simulink model "BESS_asset"  (R2026a)
settings: Solver=ode4  StopTime=inf  FixedStep=Tsim
model workspace (MATLAB code in the model file):
  | % Defaults for standalone use. In HPP.slx each instance k gets p.bess.ap(k).
  | pDefault = HPP_parameters();
  | ap   = pDefault.bess.ap(1);   % asset arguments (incl. controller par)
  | Tsim = pDefault.sim.Ts;
  | clear pDefault
libraries: sl_discontinuities x1
Description:
  | BESS asset: BESS_ctrl (asset controller) + generator / converter model (WT: IEC 61400-27-1 Type 4 generator system; PV, BESS: WECC REGC_A) feeding a current source along the angle of the controller's PLL. Per unit on the asset rating (voltage on the nominal voltage). Argument ap = p.bess.ap(k).
settings Model: ParameterArgumentNames=ap  Creator=kjaer  LastModifiedBy=kjaer

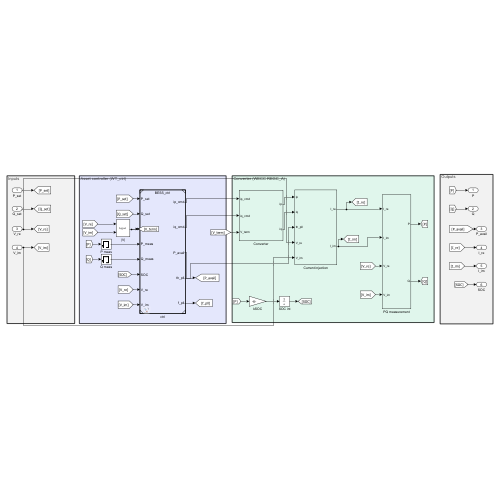
[thumbnail: Simulink's stored preview of the top-level diagram]
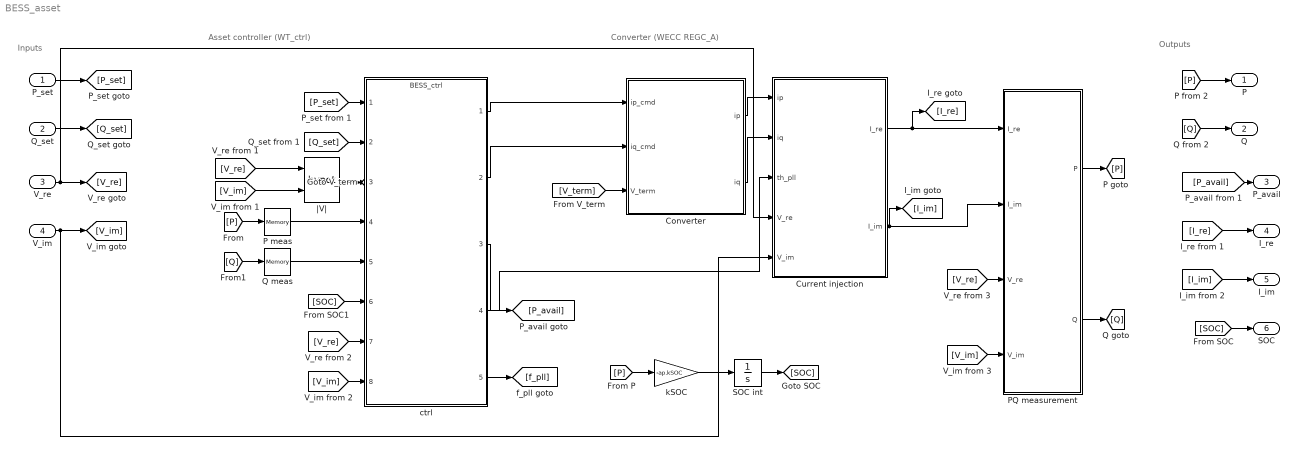
== system BESS_asset ==
  note: Outputs
  note: Converter (WECC REGC_A)
  note: Asset controller (WT_ctrl)
  note: Inputs
  P_set : Inport  OutDataTypeStr=double  PortDimensions=1
  Q_set : Inport  Port=2  OutDataTypeStr=double  PortDimensions=1
  V_re : Inport  Port=3  OutDataTypeStr=double  PortDimensions=1
  V_im : Inport  Port=4  OutDataTypeStr=double  PortDimensions=1
  Converter : Subsystem  Description=Converter (WECC REGC_A)
  Current injection : Subsystem  Description=Converter model, chosen per run by p.conv.type: Current source (1, RMS: I = (ip - j iq) e^(j th_pll)) or Averaged (2: inner dq current loop, LCL filter, DC link; params/converterParameters.m).
  P meas : Memory
  PQ measurement : Subsystem  Description=PQ measurement: P + jQ = V conj(I)
  Q meas : Memory
  SOC int : Integrator  InitialCondition=ap.SOC0
  ctrl : ModelReference  ModelNameDialog=BESS_ctrl  ParameterArgumentNames=par  ParameterArgumentValues=ap.ctrl  UsingDefaultArgumentValue=0  SimulationMode=Normal  ModelReferenceVersion=1.1
  kSOC : Gain  Gain=-ap.kSOC
  |V| : Math  Operator=hypot
  P : Outport  OutDataTypeStr=double
  Q : Outport  Port=2  OutDataTypeStr=double
  P_avail : Outport  Port=3  OutDataTypeStr=double
  I_re : Outport  Port=4  OutDataTypeStr=double
  I_im : Outport  Port=5  OutDataTypeStr=double
  SOC : Outport  Port=6  OutDataTypeStr=double
  wires:
  [Q] -> Q meas/1
  [P] -> P meas/1
  [I_im] -> I_im/1
  [I_re] -> I_re/1
  [P_avail] -> P_avail/1
  [Q] -> Q/1
  [P] -> P/1
  [V_im] -> PQ measurement/4(V_im)
  [V_re] -> PQ measurement/3(V_re)
  Current injection/2(I_im) -> [I_im], PQ measurement/2(I_im)
  Current injection/1(I_re) -> [I_re], PQ measurement/1(I_re)
  ctrl/3 -> [P_avail]
  ctrl/4 -> Current injection/3(th_pll)
  Converter/2(iq) -> Current injection/2(iq)
  Converter/1(ip) -> Current injection/1(ip)
  ctrl/2 -> Converter/2(iq_cmd)
  ctrl/1 -> Converter/1(ip_cmd)
  ctrl/5 -> [f_pll]
  [V_im] -> ctrl/8
  [V_re] -> ctrl/7
  Q meas/1 -> ctrl/5
  P meas/1 -> ctrl/4
  |V|/1 -> ctrl/3, [V_term]
  [Q_set] -> ctrl/2
  [P_set] -> ctrl/1
  PQ measurement/2(Q) -> [Q]
  PQ measurement/1(P) -> [P]
  [V_im] -> |V|/2
  [V_re] -> |V|/1
  V_im/1 -> [V_im], Current injection/5(V_im)
  V_re/1 -> [V_re], Current injection/4(V_re)
  Q_set/1 -> [Q_set]
  P_set/1 -> [P_set]
  [P] -> kSOC/1
  SOC int/1 -> [SOC]
  [SOC] -> SOC/1
  [SOC] -> ctrl/6
  [V_term] -> Converter/3(V_term)
  kSOC/1 -> SOC int/1

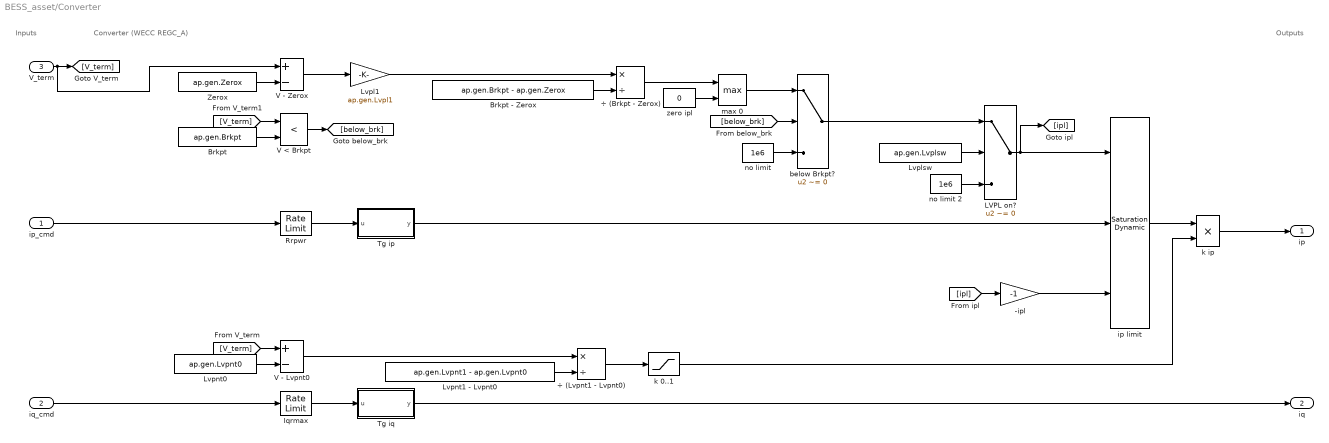
== system BESS_asset/Converter ==
  note: Inputs
  note: Converter (WECC REGC_A)
  note: Outputs
  ip_cmd : Inport  OutDataTypeStr=double  PortDimensions=1
  iq_cmd : Inport  Port=2  OutDataTypeStr=double  PortDimensions=1
  V_term : Inport  Port=3  OutDataTypeStr=double  PortDimensions=1
  -ipl : Gain  Gain=-1
  Brkpt : Constant  Value=ap.gen.Brkpt
  Brkpt - Zerox : Constant  Value=ap.gen.Brkpt - ap.gen.Zerox
  Iqrmax : RateLimiter  RisingSlewLimit=ap.gen.Iqrmax  FallingSlewLimit=ap.gen.Iqrmin  SampleTimeMode=inherited
  LVPL on? : Switch  Criteria=u2 ~= 0  SaturateOnIntegerOverflow=off  InputSameDT=off
  Lvpl1 : Gain  Gain=ap.gen.Lvpl1
  Lvplsw : Constant  Value=ap.gen.Lvplsw
  Lvpnt0 : Constant  Value=ap.gen.Lvpnt0
  Lvpnt1 - Lvpnt0 : Constant  Value=ap.gen.Lvpnt1 - ap.gen.Lvpnt0
  Rrpwr : RateLimiter  RisingSlewLimit=ap.gen.Rrpwr  FallingSlewLimit=-1e6  SampleTimeMode=inherited
  Tg ip : Subsystem  Description=first-order lag Tg; bypassed with the averaged converter (ap.conv.type = 2)
      mask Display: disp('1 / (Tg s + 1)')
  Tg iq : Subsystem  Description=first-order lag Tg; bypassed with the averaged converter (ap.conv.type = 2)
      mask Display: disp('1 / (Tg s + 1)')
  V - Lvpnt0 : Sum  Inputs=+-
  V - Zerox : Sum  Inputs=+-
  V < Brkpt : RelationalOperator  Operator=<  OutDataTypeStr=boolean  RndMeth=Simplest  InputSameDT=off
  Zerox : Constant  Value=ap.gen.Zerox
  below Brkpt? : Switch  Criteria=u2 ~= 0  SaturateOnIntegerOverflow=off  InputSameDT=off
  ip limit : sl_discontinuities/Saturation Dynamic  OutMin=[]  OutMax=[]  OutDataTypeStr=Inherit: Same as second input  OutDataType=fixdt(1, 16)  OutScaling=2^-10  DoSatur=off
      settings: LibrarySourceBlock=|
      | simulink/Discontinuities/Saturation
      | Dynamic
  k 0..1 : Saturate  UpperLimit=1  LowerLimit=0
  k ip : Product
  max 0 : MinMax  Function=max  Inputs=2
  no limit : Constant  Value=1e6
  no limit 2 : Constant  Value=1e6
  zero ipl : Constant  Value=0
  ÷ (Brkpt - Zerox) : Product  Inputs=*/
  ÷ (Lvpnt1 - Lvpnt0) : Product  Inputs=*/
  ip : Outport  OutDataTypeStr=double
  iq : Outport  Port=2  OutDataTypeStr=double
  wires:
  [ipl] -> -ipl/1
  V < Brkpt/1 -> [below_brk]
  [below_brk] -> below Brkpt?/2
  V_term/1 -> [V_term], V - Zerox/1
  [V_term] -> V - Lvpnt0/1
  [V_term] -> V < Brkpt/1
  -ipl/1 -> ip limit/3
  Brkpt - Zerox/1 -> ÷ (Brkpt - Zerox)/2
  Brkpt/1 -> V < Brkpt/2
  Iqrmax/1 -> Tg iq/1(u)
  Lvpl1/1 -> ÷ (Brkpt - Zerox)/1
  Lvplsw/1 -> LVPL on?/2
  Lvpnt0/1 -> V - Lvpnt0/2
  Lvpnt1 - Lvpnt0/1 -> ÷ (Lvpnt1 - Lvpnt0)/2
  Rrpwr/1 -> Tg ip/1(u)
  Tg ip/1(y) -> ip limit/2
  Tg iq/1(y) -> iq/1
  V - Lvpnt0/1 -> ÷ (Lvpnt1 - Lvpnt0)/1
  V - Zerox/1 -> Lvpl1/1
  Zerox/1 -> V - Zerox/2
  below Brkpt?/1 -> LVPL on?/1
  ip limit/1 -> k ip/1
  ip_cmd/1 -> Rrpwr/1
  iq_cmd/1 -> Iqrmax/1
  k 0..1/1 -> k ip/2
  k ip/1 -> ip/1
  max 0/1 -> below Brkpt?/1
  no limit 2/1 -> LVPL on?/3
  no limit/1 -> below Brkpt?/3
  zero ipl/1 -> max 0/2
  ÷ (Brkpt - Zerox)/1 -> max 0/1
  ÷ (Lvpnt1 - Lvpnt0)/1 -> k 0..1/1
  LVPL on?/1 -> ip limit/1, [ipl]

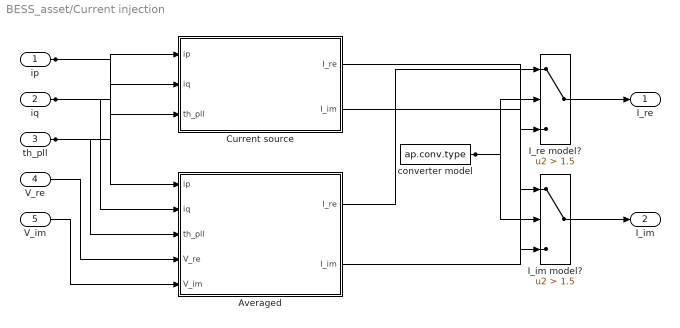
== system BESS_asset/Current injection ==
  ip : Inport
  iq : Inport  Port=2
  th_pll : Inport  Port=3
  V_re : Inport  Port=4
  V_im : Inport  Port=5
  Averaged : Subsystem  Description=Averaged converter: inner dq current loop in the PLL frame, LCL filter, DC link, angle-preserving current limit (params/converterParameters.m)  TreatAsAtomicUnit=on  SystemSampleTime=Tsim
  Current source : Subsystem  Description=Current injection along the PLL angle: I = (ip - j iq) e^(j th)
  I_im model? : Switch  Criteria=u2 > Threshold  Threshold=1.5  SaturateOnIntegerOverflow=off  InputSameDT=off
  I_re model? : Switch  Criteria=u2 > Threshold  Threshold=1.5  SaturateOnIntegerOverflow=off  InputSameDT=off
  converter model : Constant  Value=ap.conv.type
  I_re : Outport
  I_im : Outport  Port=2
  wires:
  I_re model?/1 -> I_re/1
  converter model/1 -> I_re model?/2, I_im model?/2
  I_im model?/1 -> I_im/1
  ip/1 -> Averaged/1(ip), Current source/1(ip)
  iq/1 -> Averaged/2(iq), Current source/2(iq)
  th_pll/1 -> Averaged/3(th_pll), Current source/3(th_pll)
  V_re/1 -> Averaged/4(V_re)
  V_im/1 -> Averaged/5(V_im)
  Averaged/1(I_re) -> I_re model?/1
  Current source/1(I_re) -> I_re model?/3
  Averaged/2(I_im) -> I_im model?/1
  Current source/2(I_im) -> I_im model?/3

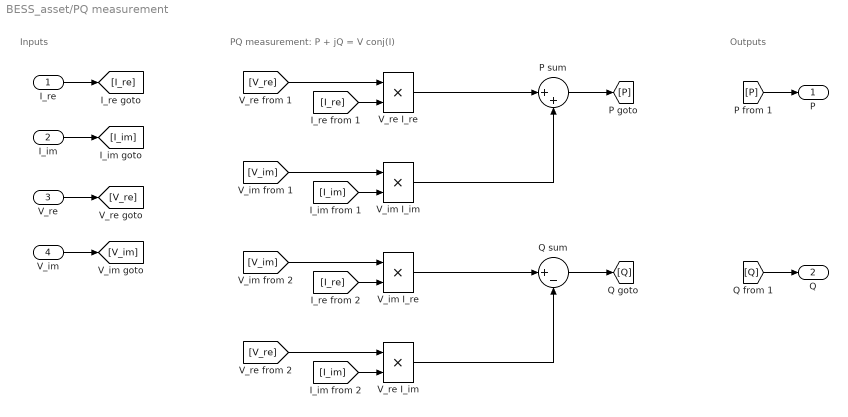
== system BESS_asset/PQ measurement ==
  note: Inputs
  note: PQ measurement: P + jQ = V conj(I)
  note: Outputs
  I_re : Inport  OutDataTypeStr=double  PortDimensions=1
  I_im : Inport  Port=2  OutDataTypeStr=double  PortDimensions=1
  V_re : Inport  Port=3  OutDataTypeStr=double  PortDimensions=1
  V_im : Inport  Port=4  OutDataTypeStr=double  PortDimensions=1
  P sum : Sum  Inputs=|++
  Q sum : Sum  Inputs=|+-
  V_im I_im : Product
  V_im I_re : Product
  V_re I_im : Product
  V_re I_re : Product
  P : Outport  OutDataTypeStr=double
  Q : Outport  Port=2  OutDataTypeStr=double
  wires:
  I_re/1 -> [I_re]
  I_im/1 -> [I_im]
  V_re/1 -> [V_re]
  V_im/1 -> [V_im]
  [V_re] -> V_re I_re/1
  [I_re] -> V_re I_re/2
  V_re I_re/1 -> P sum/1
  P sum/1 -> [P]
  [V_im] -> V_im I_im/1
  [I_im] -> V_im I_im/2
  V_im I_im/1 -> P sum/2
  [V_im] -> V_im I_re/1
  [I_re] -> V_im I_re/2
  V_im I_re/1 -> Q sum/1
  Q sum/1 -> [Q]
  [V_re] -> V_re I_im/1
  [I_im] -> V_re I_im/2
  V_re I_im/1 -> Q sum/2
  [P] -> P/1
  [Q] -> Q/1

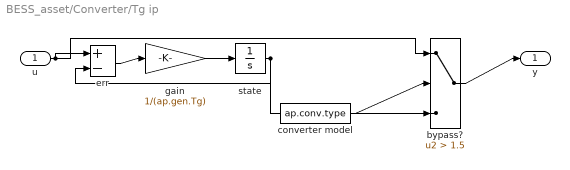
== system BESS_asset/Converter/Tg ip ==
  u : Inport
  bypass? : Switch  Criteria=u2 > Threshold  Threshold=1.5  SaturateOnIntegerOverflow=off  InputSameDT=off
  converter model : Constant  Value=ap.conv.type
  err : Sum  Inputs=+-
  gain : Gain  Gain=1/(ap.gen.Tg)
  state : Integrator
  y : Outport
  wires:
  u/1 -> err/1, bypass?/1
  err/1 -> gain/1
  gain/1 -> state/1
  state/1 -> bypass?/3, err/2
  converter model/1 -> bypass?/2
  bypass?/1 -> y/1

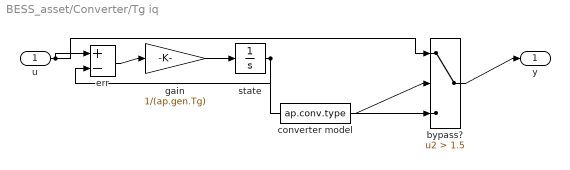
== system BESS_asset/Converter/Tg iq ==
  u : Inport
  bypass? : Switch  Criteria=u2 > Threshold  Threshold=1.5  SaturateOnIntegerOverflow=off  InputSameDT=off
  converter model : Constant  Value=ap.conv.type
  err : Sum  Inputs=+-
  gain : Gain  Gain=1/(ap.gen.Tg)
  state : Integrator
  y : Outport
  wires:
  u/1 -> err/1, bypass?/1
  err/1 -> gain/1
  gain/1 -> state/1
  state/1 -> bypass?/3, err/2
  converter model/1 -> bypass?/2
  bypass?/1 -> y/1

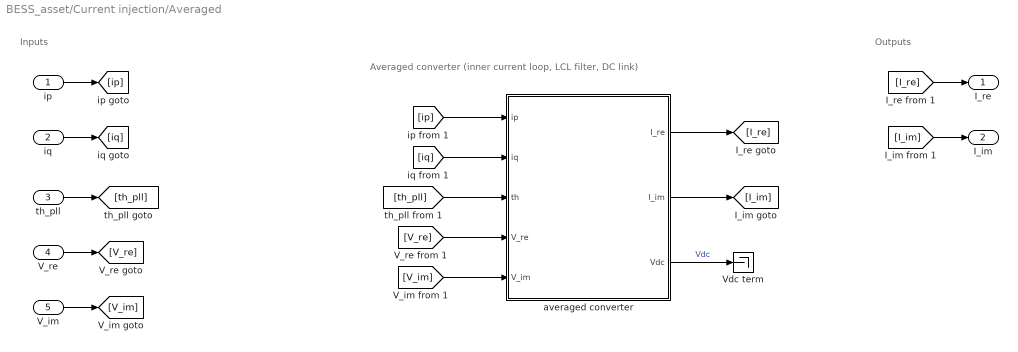
== system BESS_asset/Current injection/Averaged ==
  note: Inputs
  note: Averaged converter (inner current loop, LCL filter, DC link)
  note: Outputs
  ip : Inport  OutDataTypeStr=double  PortDimensions=1
  iq : Inport  Port=2  OutDataTypeStr=double  PortDimensions=1
  th_pll : Inport  Port=3  OutDataTypeStr=double  PortDimensions=1
  V_re : Inport  Port=4  OutDataTypeStr=double  PortDimensions=1
  V_im : Inport  Port=5  OutDataTypeStr=double  PortDimensions=1
  Vdc term : Terminator
  averaged converter : MATLAB Function  TreatAsAtomicUnit=on
  I_re : Outport  OutDataTypeStr=double
  I_im : Outport  Port=2  OutDataTypeStr=double
  wires:
  ip/1 -> [ip]
  iq/1 -> [iq]
  th_pll/1 -> [th_pll]
  V_re/1 -> [V_re]
  V_im/1 -> [V_im]
  [ip] -> averaged converter/1(ip)
  [iq] -> averaged converter/2(iq)
  [th_pll] -> averaged converter/3(th)
  [V_re] -> averaged converter/4(V_re)
  [V_im] -> averaged converter/5(V_im)
  averaged converter/3(Vdc) -> Vdc term/1  "Vdc"
  averaged converter/1(I_re) -> [I_re]
  averaged converter/2(I_im) -> [I_im]
  [I_re] -> I_re/1
  [I_im] -> I_im/1

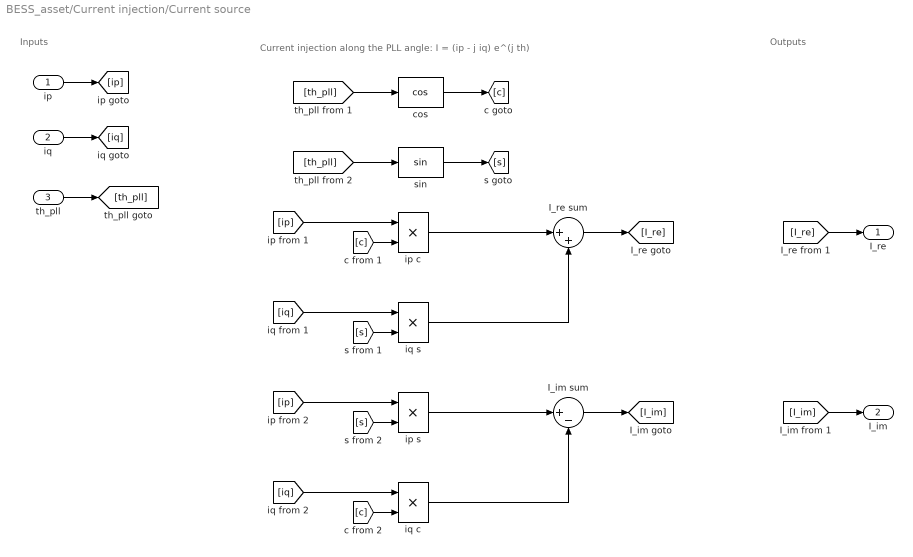
== system BESS_asset/Current injection/Current source ==
  note: Inputs
  note: Current injection along the PLL angle: I = (ip - j iq) e^(j th)
  note: Outputs
  ip : Inport  OutDataTypeStr=double  PortDimensions=1
  iq : Inport  Port=2  OutDataTypeStr=double  PortDimensions=1
  th_pll : Inport  Port=3  OutDataTypeStr=double  PortDimensions=1
  I_im sum : Sum  Inputs=|+-
  I_re sum : Sum  Inputs=|++
  cos : Trigonometry  Operator=cos
  ip c : Product
  ip s : Product
  iq c : Product
  iq s : Product
  sin : Trigonometry
  I_re : Outport  OutDataTypeStr=double
  I_im : Outport  Port=2  OutDataTypeStr=double
  wires:
  ip/1 -> [ip]
  iq/1 -> [iq]
  th_pll/1 -> [th_pll]
  [th_pll] -> cos/1
  cos/1 -> [c]
  [th_pll] -> sin/1
  sin/1 -> [s]
  [ip] -> ip c/1
  [c] -> ip c/2
  ip c/1 -> I_re sum/1
  I_re sum/1 -> [I_re]
  [iq] -> iq s/1
  [s] -> iq s/2
  iq s/1 -> I_re sum/2
  [ip] -> ip s/1
  [s] -> ip s/2
  ip s/1 -> I_im sum/1
  I_im sum/1 -> [I_im]
  [iq] -> iq c/1
  [c] -> iq c/2
  iq c/1 -> I_im sum/2
  [I_re] -> I_re/1
  [I_im] -> I_im/1

== matlab function BESS_asset/Current injection/Averaged/averaged converter ==
  data: ip input; I_re output; iq input; th input; V_re input; V_im input; I_im output; Vdc output; ap parameter
function [I_re, I_im, Vdc] = avg_converter(ip, iq, th, V_re, V_im, ap)
%#codegen
c = ap.conv;
persistent x xi xdc w ps
if c.type < 1.5                        % current source selected: nothing to do
    I_re = 0;  I_im = 0;  Vdc = c.Vdc0;
    return
end
vg = complex(V_re, V_im);
e  = complex(cos(th), sin(th));        % PLL frame -> common frame
ec = conj(e);
i2r = complex(ip, -iq);                % grid current reference, PLL frame
pstar = real(vg * conj(i2r * e));      % commanded power (source behind the DC link)
if isempty(x)
    % start in steady state at the first terminal voltage
    i2 = i2r * e;
    vC = vg + complex(c.R2, c.L2) * i2;
    i1 = i2 + 1j * c.Cf * vC;
    x  = [i1; vC; i2];
    xi = c.R1 * i1 * ec;
    xdc = 0;  w = c.Vdc0^2;  ps = pstar;
end
Ad = complex(c.AdRe, c.AdIm);  Bd = complex(c.BdRe, c.BdIm);
w0ref = c.Vdc0^2;
for k = 1:c.n
    i1 = x(1);  vn = x(2) + c.RdUsed * (x(1) - x(3));
    i1d = i1 * ec;  vnd = vn * ec;      % PLL frame
    % DC voltage loop (PI on Vdc^2): extra active current
    err = w - w0ref;
    dP = c.kpDC * err + xdc;
    % current reference: grid current + DC correction + capacitor current
    i1r = i2r + dP / max(abs(vnd), 0.1) + 1j * c.Cf * vnd;
    m = abs(i1r);  lim = m > c.Imax;
    if lim, i1r = i1r * (c.Imax / m); end   % angle-preserving limit
    if ~lim, xdc = xdc + c.kiDC * c.h * err; end
    % current PI with decoupling and feed-forward of vn
    ei = i1r - i1d;
    v = vnd + 1j * c.L1 * i1d + c.kp * ei + xi;
    vmax = c.mMax * sqrt(max(w, 0));
    if abs(v) > vmax
        v = v * (vmax / abs(v));         % modulation limit, no integration
    else
        xi = xi + c.ki * c.h * ei;
    end
    vc = v * e;
    % DC link: source power through a lag, converter power out; chopper
    pc = real(vc * conj(i1));
    ps = ps + (c.h / c.Tsrc) * (pstar - ps);
    w = min(max(w + c.h * (ps - pc) / c.Hdc, 0.01), c.Vchop^2);
    % LCL filter, exact over the sub-step
    x = Ad * x + Bd * [vc; vg];
end
I_re = real(x(3));  I_im = imag(x(3));
Vdc = sqrt(w);
end
